simulink model "OpenLoopDriveTest"  (R2026b)
settings: Solver=FixedStepDiscrete  StopTime=openLoopTestCfg.Duration  FixedStep=openLoopCfg.Ts
PostLoadFcn:
  | addpath(fullfile(fileparts(get_param(bdroot,'FileName')),'..','build_process'));initialize_open_loop_drive_test(bdroot);
model workspace (MAT data in the model file):
  openLoopCfg.Ts = 6.25e-05
  openLoopCfg.Kind = 1
  openLoopCfg.MaximumFrequency = 80
  openLoopCfg.FrequencySlew = 40
  openLoopCfg.ObserveTime = 0.05
  openLoopCfg.StartVoltageMaximum = 0.25
  openLoopCfg.StartCurrentMaximum = 0.2
  openLoopCfg.ObserveTimeout = 0.5
  openLoopCfg.AlignTime = 0.25
  openLoopCfg.AlignRampTime = 0.1
  openLoopCfg.AlignAmplitude = 2
  openLoopCfg.RunAmplitude = 3
  openLoopCfg.AmplitudeSlew = 40
  openLoopCfg.VfSlope = 0.219911485751
  openLoopCfg.VfBoost = 0.5
  openLoopCfg.VoltageFraction = 0.554256258422
  openLoopCfg.CurrentTrip = 12
  openLoopCfg.Theta0 = 0
  openLoopCfg.ObserveTicks = 800
  openLoopCfg.ObserveTimeoutTicks = 8000
  openLoopCfg.AlignTicks = 4000
  openLoopCfg.AlignRampTicks = 1600
  openLoopCfg.Vector = [6.25e-05; 1; 80; 40; 800; 0.25; 0.2; 8000; 4000; 1600; 2; 3; 40; 0.219911485751; 0.5; 0.554256258422; 12; 0]
  openLoopCfg.State0 = [0; 0; 0; 0; 0; 0; 0; 0]
  openLoopTestCfg.Duration = 0.8
  openLoopTestCfg.Frequency = 20
  openLoopTestCfg.BusVoltage = 48
  openLoopTestCfg.Current = 0
  openLoopTestCfg.TerminalVoltage = 0
  openLoopTestCfg.ValidationTs = 0.0001
  openLoopTestCfg.ObserveTime = 0.01
  openLoopTestCfg.ObserveTimeout = 0.08
  openLoopTestCfg.AlignTime = 0.08
  openLoopTestCfg.AlignRampTime = 0.04
  openLoopTestCfg.FaultTime = 0.4
  openLoopTestCfg.ClearEndTime = 0.41
  openLoopTestCfg.LimitFrequency = 120
  openLoopTestCfg.LimitSlew = 200
  openLoopTestCfg.LimitedBus = 6
  openLoopTestCfg.MovingTerminal = 4
  openLoopTestCfg.VfSlope = 1
  openLoopTestCfg.AlignVoltage = 0.5
  openLoopTestCfg.PhaseTolerance = 1e-10
  testStim.time = []
  testStim.signals.values = [20 20 20 20 20 20 20 20 20 20 20 20 ... (76806 elements, 12801x6)]
  testStim.signals.dimensions = 6
libraries: OpenLoopDrive x1
settings Model: Creator=24322  LastModifiedBy=24322

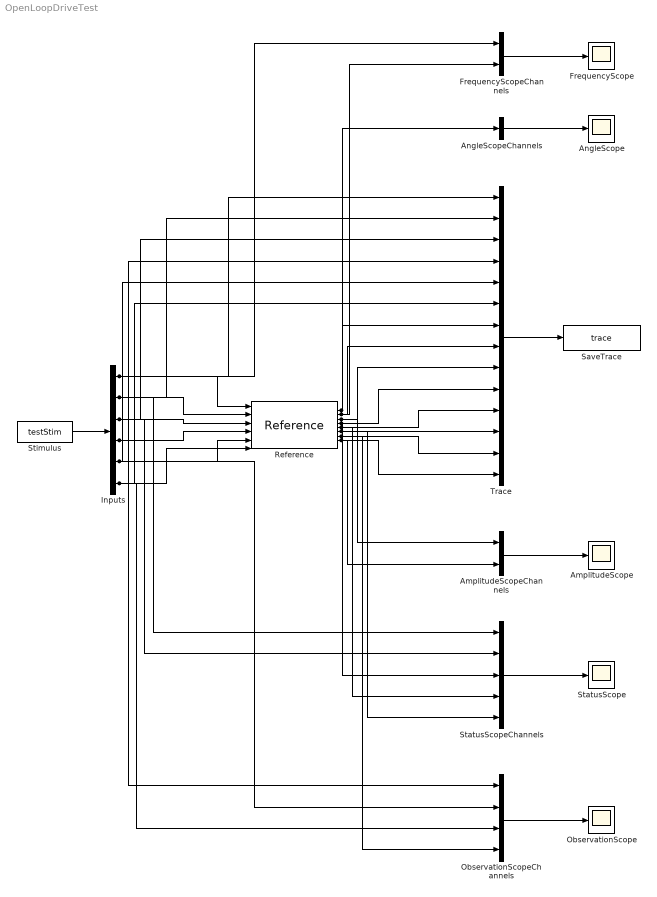
== system OpenLoopDriveTest ==
  AmplitudeScope : Scope
  AmplitudeScopeChannels : Mux  Inputs=2
  AngleScope : Scope
  AngleScopeChannels : Mux  Inputs=1
  FrequencyScope : Scope
  FrequencyScopeChannels : Mux  Inputs=2
  Inputs : Demux  Outputs=6
  ObservationScope : Scope
  ObservationScopeChannels : Mux
  Reference : OpenLoopDrive/Reference  openLoopCfg=openLoopCfg
  SaveTrace : ToWorkspace  VariableName=trace  SaveFormat=Structure With Time  SampleTime=openLoopCfg.Ts
  StatusScope : Scope
  StatusScopeChannels : Mux  Inputs=5
  Stimulus : FromWorkspace  VariableName=testStim  SampleTime=openLoopCfg.Ts  Interpolate=off  OutputAfterFinalValue=Holding final value
  Trace : Mux  Inputs=14
  wires:
  ObservationScopeChannels/1 -> ObservationScope/1
  StatusScopeChannels/1 -> StatusScope/1
  AmplitudeScopeChannels/1 -> AmplitudeScope/1
  FrequencyScopeChannels/1 -> FrequencyScope/1
  AngleScopeChannels/1 -> AngleScope/1
  Reference/8 -> Trace/14, AmplitudeScopeChannels/2
  Reference/7 -> Trace/13, ObservationScopeChannels/4
  Reference/6 -> Trace/12, StatusScopeChannels/5
  Reference/5 -> Trace/11, StatusScopeChannels/4
  Reference/4 -> Trace/10, StatusScopeChannels/3
  Reference/3 -> Trace/9, AmplitudeScopeChannels/1
  Reference/2 -> Trace/8, FrequencyScopeChannels/2
  Reference/1 -> Trace/7, AngleScopeChannels/1
  Inputs/6 -> Trace/6, Reference/6, ObservationScopeChannels/3
  Inputs/5 -> Reference/5, Trace/5, ObservationScopeChannels/2
  Inputs/4 -> Trace/4, Reference/4, ObservationScopeChannels/1
  Inputs/3 -> Trace/3, Reference/3, StatusScopeChannels/2
  Inputs/2 -> Reference/2, Trace/2, StatusScopeChannels/1
  Inputs/1 -> Trace/1, Reference/1, FrequencyScopeChannels/1
  Trace/1 -> SaveTrace/1
  Stimulus/1 -> Inputs/1
